simulink model "Motorcycle_Sym"  (R2022a)
settings: Solver=FixedStepAuto  StartTime=0.0  StopTime=inf  RelTol=1e-3  EnableMultiTasking=on
undefined symbols (not defined in the file): DiscIntNeverNeededParam
libraries: arduinomotorcarrierlib x4, simulink x4, arduinosensorlib x2, arduinolib x1
settings Model: SimulationMode=external  ExtModeTrigDuration=2  Creator=gandr  LastModifiedBy=ix_andrei
settings SolverCC: AutoInsertRateTranBlk=on
settings OptimizationCC: EnhancedBackFolding=on  PassReuseOutputArgsAs=Individual arguments  ZeroExternalMemoryAtStartup=off  ZeroInternalMemoryAtStartup=off  MaxStackSize=64  OptimizeBlockOrder=speed  DifferentSizesBufferReuse=on  OptimizationCustomize=off  EfficientTunableParamExpr=on
settings DebuggingCC: MultiTaskRateTransMsg=warning  ParameterTunabilityLossMsg=error  UnconnectedInputMsg=warning  UnconnectedOutputMsg=warning  UnconnectedLineMsg=warning
settings HardwareCC: ProdBitPerPointer=32  ProdBitPerSizeT=32  ProdBitPerPtrDiffT=32  ProdLargestAtomicInteger=Long  ProdLargestAtomicFloat=Double  ProdWordSize=32  ProdHWDeviceType=ARM Compatible->ARM Cortex  UseEmbeddedCoderFeatures=off  UseSimulinkCoderFeatures=off
settings SFSimCC: MATLABDynamicMemAlloc=off
settings RTWCC: SystemTargetFile=ert.tlc  HardwareBoard=Arduino MKR1000  TemplateMakefile=ert_default_tmf  Toolchain=Arduino ARM  BuildConfiguration=Faster Runs  DLArmComputeVersion=19.05
settings CodeAppCC: ForceParamTrailComments=on  IgnoreCustomStorageClasses=off  OperatorAnnotations=on  SimulinkDataObjDesc=on  SFDataObjDesc=on  MangleLength=10  InsertBlockDesc=on
settings ERTTargetCC: SupportContinuousTime=on  SupportNonInlinedSFcns=on  SupportVariableSizeSignals=on  ExtModeTransport=3  ExtModeStaticAlloc=on  ExtModeStaticAllocSize=8192  ExtModeMexFile=ext_xcp  ExtModeIntrfLevel=Level2 - Open

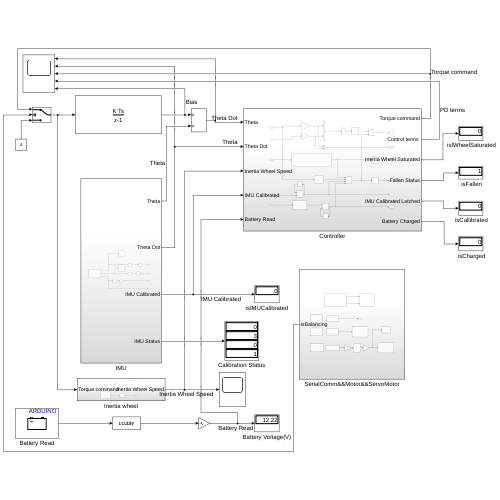
[thumbnail: Simulink's stored preview of the top-level diagram]
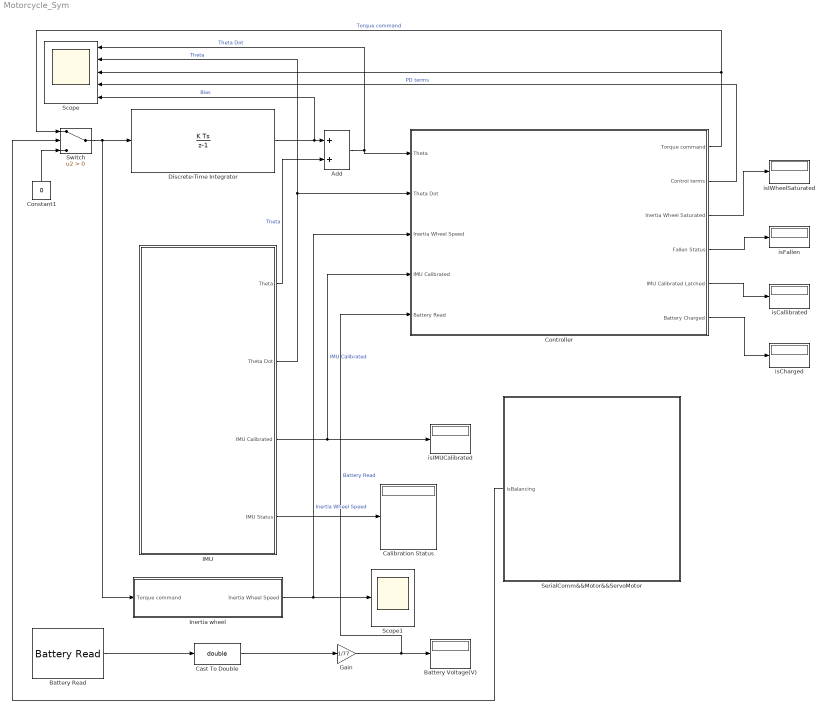
== system Motorcycle_Sym ==
  " isCallibrated" : Display
  " isCharged" : Display
  " isFallen" : Display
  " isIWheelSaturated" : Display
  Add : Sum
  Battery Read : arduinomotorcarrierlib/Battery Read  SlaveAddress=uint8( hex2dec( '66' ) )  blockPlatform=ARDUINO  SampleTime=0.1
      settings: SourceProductBaseCode=ARDUINO
  Battery Voltage(V) : Display
  Calibration Status : Display
  Cast To Double : DataTypeConversion  OutDataTypeStr=double  SaturateOnIntegerOverflow=off  RndMeth=Floor
  Constant1 : Constant  Value=0
  Controller : Subsystem
  Discrete-Time Integrator : DiscreteIntegrator  gainval=1  SampleTime=-1  ICPrevOutput=DiscIntNeverNeededParam  ICPrevScaledInput=DiscIntNeverNeededParam
  Gain : Gain  Gain=1/77
  IMU : Subsystem
  Inertia wheel : Subsystem
  Scope : Scope  NumInputPorts=5
  Scope1 : Scope
  SerialComm&&Motor&&ServoMotor : Subsystem
      settings: PortSchema="{\"entries\":[{\"content\":{\"sides\":[{\"content\":{\"connectorIds\":[\"Out1\"]},\"type\":\"ConnectorPlacement.EquallySpacedRectSide\",\"uuid\":\"a54661e8-14d7-4d42-8b3e-50e0f1fc35d2\"},{\"content\":{\"connectorIds\":[],\"side\":\"RIGHT\"},\"type\":\"ConnectorPlacement.EquallySpacedRectSide\",\"uuid\":\"73e1e260-bb35-49f7-9715-a15b09c38e42\"},{\"content\":{\"connectorIds\":[],\"side\":\"TOP\"},\"type\":\"ConnectorPlacement.EquallySpacedRectSide\",\"uuid\":\"b46773ac-ef8a-4d86-b290-907da0b08aad\"}]},\"type\":\"ConnectorPlacement.EquallySpacedConnector\",\"uuid\":\"c2ad3030-f234-4b50-94ae-35547127ef1c\"}],\"packageUris\":[\"http://schema.mathworks.com/mf0/Connector/R2020b\"],\"version\":\"1.0\"}"
  Switch : Switch  Criteria=u2 > Threshold  SaturateOnIntegerOverflow=off  InputSameDT=off
  isIMUCalibrated : Display
  wires:
  Discrete-Time Integrator/1 -> Scope/5, Add/1  "Bias"
  Constant1/1 -> Switch/3
  Controller/3(Inertia Wheel Saturated) -> " isIWheelSaturated"/1
  Controller/5(IMU Calibrated Latched) -> " isCallibrated"/1
  Controller/4(Fallen Status) -> " isFallen"/1
  Controller/2("Control terms ") -> Scope/4  "PD terms"
  Controller/1(Torque command) -> Scope/3, Switch/1  "Torque command"
  Cast To Double/1 -> Gain/1
  Controller/6(Battery Charged) -> " isCharged"/1
  IMU/4(IMU Status) -> Calibration Status/1
  Battery Read/1 -> Cast To Double/1
  IMU/1(Theta) -> Add/2  "Theta"
  Add/1 -> Controller/1(Theta), Scope/1  "Theta Dot"
  Inertia wheel/1(Inertia Wheel Speed) -> Scope1/1, Controller/3(Inertia Wheel Speed)  "Inertia Wheel Speed"
  Switch/1 -> Discrete-Time Integrator/1, Inertia wheel/1(Torque command)
  Gain/1 -> Battery Voltage(V)/1, Controller/5(Battery Read)  "Battery Read"
  IMU/3(IMU Calibrated) -> isIMUCalibrated/1, Controller/4(IMU Calibrated)  "IMU Calibrated"
  IMU/2(Theta Dot) -> Controller/2(Theta Dot), Scope/2  "Theta"
  SerialComm&&Motor&&ServoMotor/1(isBalancing) -> Switch/2

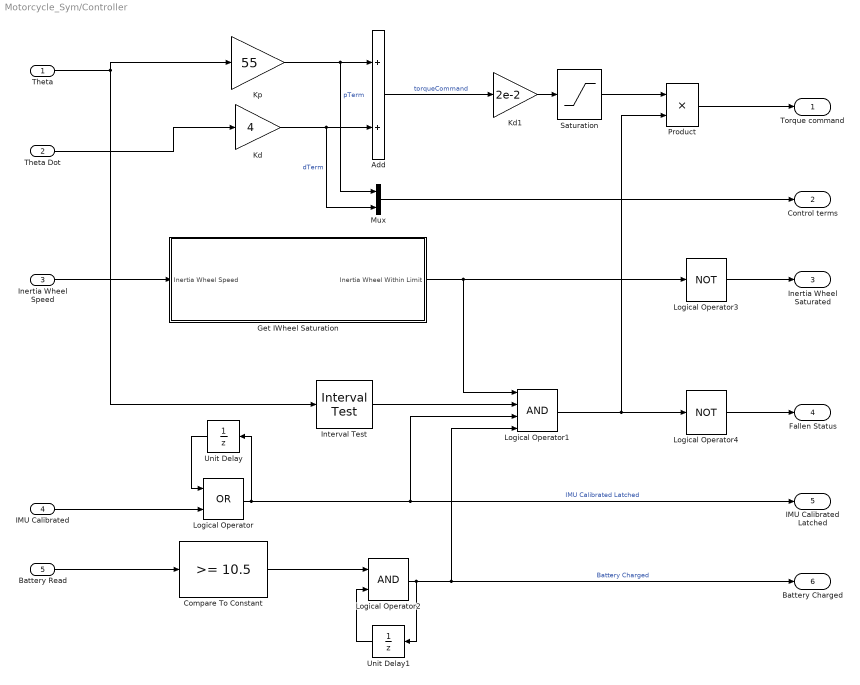
== system Motorcycle_Sym/Controller ==
  Theta : Inport
  Theta Dot : Inport  Port=2
  Inertia Wheel Speed : Inport  Port=3
  IMU Calibrated : Inport  Port=4
  Battery Read : Inport  Port=5
  Add : Sum
  Compare To Constant : simulink/Logic and Bit Operations/Compare To Constant  relop=>=  const=10.5  OutDataTypeStr=boolean
  Get IWheel Saturation : Subsystem
  Interval Test : simulink/Logic and Bit Operations/Interval Test  IntervalClosedRight=on  uplimit=12  IntervalClosedLeft=on  lowlimit=-12  OutDataTypeStr=boolean
  Kd : Gain  Gain=4
  Kd1 : Gain  Gain=2e-2
  Kp : Gain  Gain=55
  Logical Operator : Logic  Operator=OR  AllPortsSameDT=off  OutDataTypeStr=boolean
  Logical Operator1 : Logic  Inputs=4  AllPortsSameDT=off  OutDataTypeStr=boolean
  Logical Operator2 : Logic  AllPortsSameDT=off  OutDataTypeStr=boolean
  Logical Operator3 : Logic  Operator=NOT  AllPortsSameDT=off  OutDataTypeStr=boolean
  Logical Operator4 : Logic  Operator=NOT  AllPortsSameDT=off  OutDataTypeStr=boolean
  Mux : Mux  Inputs=2
  Product : Product
  Saturation : Saturate  UpperLimit=0.7  LowerLimit=-0.7
  Unit Delay : UnitDelay  SampleTime=-1  HasFrameUpgradeWarning=on
  Unit Delay1 : UnitDelay  InitialCondition=1  SampleTime=-1  HasFrameUpgradeWarning=on
  Torque command : Outport
  "Control terms " : Outport  Port=2
  Inertia Wheel Saturated : Outport  Port=3
  Fallen Status : Outport  Port=4
  IMU Calibrated Latched : Outport  Port=5
  Battery Charged : Outport  Port=6
  wires:
  Unit Delay1/1 -> Logical Operator2/2
  Logical Operator1/1 -> Product/2, Logical Operator4/1
  Logical Operator/1 -> IMU Calibrated Latched/1, Logical Operator1/3, Unit Delay/1  "IMU Calibrated Latched"
  Theta/1 -> Kp/1, Interval Test/1
  Product/1 -> Torque command/1
  Logical Operator2/1 -> Unit Delay1/1, Battery Charged/1, Logical Operator1/4  "Battery Charged"
  Compare To Constant/1 -> Logical Operator2/1
  Get IWheel Saturation/1(Inertia Wheel Within Limit) -> Logical Operator3/1, Logical Operator1/1
  Kd1/1 -> Saturation/1
  Kd/1 -> Add/2, Mux/2  "dTerm"
  Kp/1 -> Add/1, Mux/1  "pTerm"
  Unit Delay/1 -> Logical Operator/1
  Saturation/1 -> Product/1
  Add/1 -> Kd1/1  "torqueCommand"
  Mux/1 -> "Control terms "/1
  Logical Operator4/1 -> Fallen Status/1
  Interval Test/1 -> Logical Operator1/2
  Theta Dot/1 -> Kd/1
  Logical Operator3/1 -> Inertia Wheel Saturated/1
  Inertia Wheel Speed/1 -> Get IWheel Saturation/1(Inertia Wheel Speed)
  Battery Read/1 -> Compare To Constant/1
  IMU Calibrated/1 -> Logical Operator/2

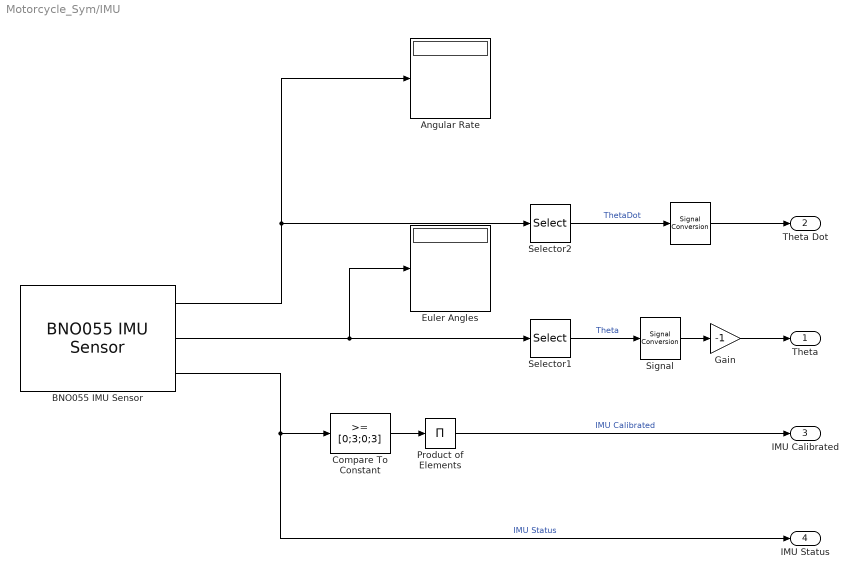
== system Motorcycle_Sym/IMU ==
  " " : SignalConversion  OverrideOpt=off
  Angular Rate : Display
  BNO055 IMU Sensor : arduinosensorlib/BNO055 IMU Sensor  SlaveAddress=0x28  OperationMode=Fusion  Accel=off  AngularRate=on  MagField=off  EulerAngles=on  Quat=off  LinearAccel=off  GravityVector=off  Status=on  AccelRange=4G  AccelBW=62.5 Hz  GyroRange=2000 dps  GyroBW=32 Hz  MagODR=10 Hz  SampleTime=0.01  blockPlatform=ARDUINO
      settings: SourceProductName=Simulink Support for Arduino Sensors
  Compare To Constant : simulink/Logic and Bit Operations/Compare To Constant  relop=>=  const=[0;3;0;3]  OutDataTypeStr=boolean
  Euler Angles : Display
  Gain : Gain  Gain=-1
  Product of Elements : Product  Inputs=*
  Selector1 : Selector  InputPortWidth=3  IndexOptions=Index vector (dialog)  Indices=2  OutputSizes=1
  Selector2 : Selector  InputPortWidth=3  IndexOptions=Index vector (dialog)  Indices=2  OutputSizes=1
  "Signal " : SignalConversion  OverrideOpt=off
  Theta : Outport  VectorParamsAs1DForOutWhenUnconnected=off
  Theta Dot : Outport  Port=2  VectorParamsAs1DForOutWhenUnconnected=off
  IMU Calibrated : Outport  Port=3  VectorParamsAs1DForOutWhenUnconnected=off
  IMU Status : Outport  Port=4  VectorParamsAs1DForOutWhenUnconnected=off
  wires:
  BNO055 IMU Sensor/2 -> Euler Angles/1, Selector1/1
  BNO055 IMU Sensor/1 -> Selector2/1, Angular Rate/1
  BNO055 IMU Sensor/3 -> IMU Status/1, Compare To Constant/1  "IMU Status"
  Compare To Constant/1 -> Product of Elements/1
  Product of Elements/1 -> IMU Calibrated/1  "IMU Calibrated"
  Selector1/1 -> "Signal "/1  "Theta"
  Gain/1 -> Theta/1
  Selector2/1 -> " "/1  "ThetaDot"
  " "/1 -> Theta Dot/1
  "Signal "/1 -> Gain/1

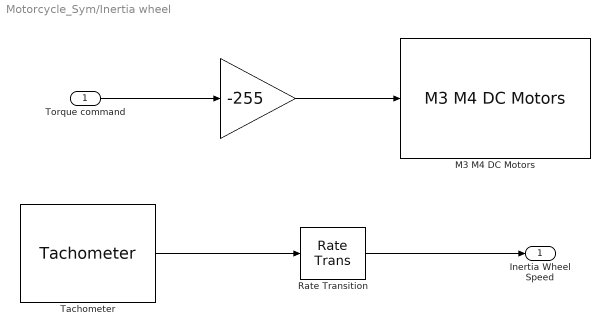
== system Motorcycle_Sym/Inertia wheel ==
  Torque command : Inport
  " " : Gain  Gain=-255
  M3 M4 DC Motors : arduinomotorcarrierlib/M3 M4 DC Motors  MotorNumber=M3  forwardPinNumber=3  reversePinNumber=2
      settings: SourceProductBaseCode=ARDUINO
  Rate Transition : RateTransition
  Tachometer : arduinosensorlib/Tachometer  PinNumber=16  InterruptMode=RISING  PulseCountperRotation=2  SampleTime=0.1  blockPlatform=ARDUINO
      settings: SourceProductBaseCode=ARDUINO
  Inertia Wheel Speed : Outport
  wires:
  Rate Transition/1 -> Inertia Wheel Speed/1
  " "/1 -> M3 M4 DC Motors/1
  Torque command/1 -> " "/1
  Tachometer/1 -> Rate Transition/1

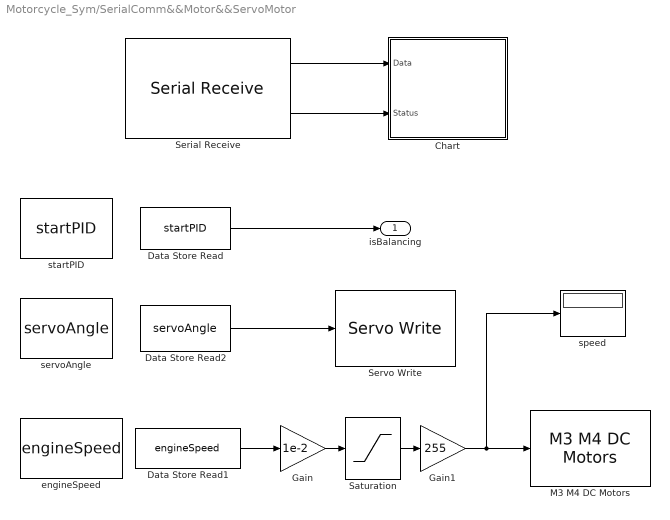
== system Motorcycle_Sym/SerialComm&&Motor&&ServoMotor ==
  Chart : Stateflow chart  TreatAsAtomicUnit=on
      settings: PortSchema="{\"entries\":[{\"content\":{\"sides\":[{\"content\":{\"connectorIds\":[\"In2\",\"In1\"]},\"type\":\"ConnectorPlacement.EquallySpacedRectSide\",\"uuid\":\"d24d2de7-555f-4848-95a1-a2290747bdbf\"},{\"content\":{\"connectorIds\":[],\"side\":\"RIGHT\"},\"type\":\"ConnectorPlacement.EquallySpacedRectSide\",\"uuid\":\"32b287f3-9753-4e37-b96d-c173438cdfd3\"},{\"content\":{\"connectorIds\":[],\"side\":\"TOP\"},\"type\":\"ConnectorPlacement.EquallySpacedRectSide\",\"uuid\":\"18668b98-b535-4338-b7b6-776d371cf657\"}]},\"type\":\"ConnectorPlacement.EquallySpacedConnector\",\"uuid\":\"e6f33e9b-cbde-4eaf-92de-13098f847cba\"}],\"packageUris\":[\"http://schema.mathworks.com/mf0/Connector/R2020b\"],\"version\":\"1.0\"}"
  Data Store Read : DataStoreRead  DataStoreName=startPID  SampleTime=0.01  IndexOptions=Index vector (dialog)  Indices=1  OutputSizes=1
  Data Store Read1 : DataStoreRead  DataStoreName=engineSpeed  SampleTime=0.01  IndexOptions=Index vector (dialog)  Indices=1  OutputSizes=1
  Data Store Read2 : DataStoreRead  DataStoreName=servoAngle  SampleTime=0.01  IndexOptions=Index vector (dialog)  Indices=1  OutputSizes=1
  Gain : Gain  Gain=1e-2
  Gain1 : Gain  Gain=255
  M3 M4 DC Motors : arduinomotorcarrierlib/M3 M4 DC Motors  MotorNumber=M4  forwardPinNumber=4  reversePinNumber=5
      settings: SourceProductBaseCode=ARDUINO
  Saturation : Saturate  UpperLimit=0.9  LowerLimit=-0.9
  Serial Receive : arduinolib/Serial Receive  isARMArch=on  portNumber=1  DataType=uint8  Datalength=2  SampleTime=0.01  showOutStatus=on  blockPlatform=arduino
      settings: SourceProductBaseCode=ARDUINO
  Servo Write : arduinomotorcarrierlib/Servo Write  SlaveAddress=uint8( hex2dec( '66' ) )  blockPlatform=ARDUINO  MotorNumber=3  MotorCarrierPWMFreq=100
      settings: SourceProductBaseCode=ARDUINO
  engineSpeed : DataStoreMemory  DataStoreName=engineSpeed  ReadBeforeWriteMsg=warning  WriteAfterWriteMsg=warning  WriteAfterReadMsg=warning  ShowAdditionalParam=off  OutMin=-100  OutMax=100  OutDataTypeStr=double
  servoAngle : DataStoreMemory  DataStoreName=servoAngle  ReadBeforeWriteMsg=warning  WriteAfterWriteMsg=warning  WriteAfterReadMsg=warning  InitialValue=108  VectorParams1D=off  ShowAdditionalParam=off  OutMin=78  OutMax=138  OutDataTypeStr=uint8
  speed : Display
  startPID : DataStoreMemory  DataStoreName=startPID  WriteAfterWriteMsg=warning  InitialValue=false  ShowAdditionalParam=off  OutDataTypeStr=boolean
  isBalancing : Outport
  wires:
  Serial Receive/1 -> Chart/2(Data)
  Data Store Read/1 -> isBalancing/1
  Data Store Read2/1 -> Servo Write/1
  Serial Receive/2 -> Chart/1(Status)
  Data Store Read1/1 -> Gain/1
  Gain/1 -> Saturation/1
  Gain1/1 -> speed/1, M3 M4 DC Motors/1
  Saturation/1 -> Gain1/1

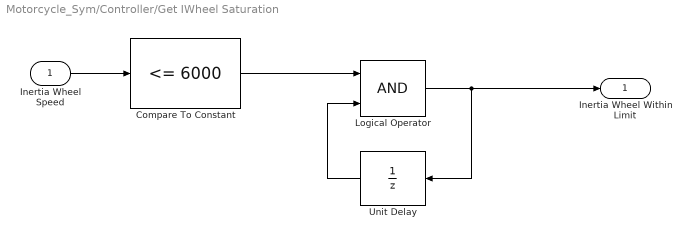
== system Motorcycle_Sym/Controller/Get IWheel Saturation ==
  Inertia Wheel Speed : Inport
  Compare To Constant : simulink/Logic and Bit Operations/Compare To Constant  relop=<=  const=6000  OutDataTypeStr=boolean
  Logical Operator : Logic  AllPortsSameDT=off  OutDataTypeStr=boolean
  Unit Delay : UnitDelay  InitialCondition=1  SampleTime=-1  HasFrameUpgradeWarning=on
  Inertia Wheel Within Limit : Outport
  wires:
  Logical Operator/1 -> Inertia Wheel Within Limit/1, Unit Delay/1
  Compare To Constant/1 -> Logical Operator/1
  Unit Delay/1 -> Logical Operator/2
  Inertia Wheel Speed/1 -> Compare To Constant/1

== stateflow chart Motorcycle_Sym/SerialComm&&Motor&&ServoMotor/Chart ==
  state idleState
  state newCommand
    if(Data(1)==0x01 && Data(2)==0x01)
    startPID = true;
    elseif(Data(1)==0x01 && Data(2)==0x00)
    startPID = false;
    elseif(Data(1)==0x02)
    engineSpeed = -double(Data(2));
    elseif(Data(1)==0x12)
    engineSpeed = double(Data(2));
    elseif(Data(1)==0x03)
    servoAngle = 0.97*uint8(Data(2))+0.03*servoAngle;
    end;
  (default) -> idleState
  idleState -> newCommand : [(Data(1) ~= 0x00) && (Status == 1)]
  newCommand -> idleState : [(Data(1) == 0x00) || (Status ~= 1)]
  data: Status input; Data input uint8 size=2; engineSpeed data_store_memory; servoAngle data_store_memory; startPID data_store_memory
